simulink model "issue2_drive_demo"  (R2024b)
settings: Solver=FixedStepDiscrete  StartTime=0.0  StopTime=1  FixedStep=.001  RelTol=1e-3
InitFcn:
  | addpath(fullfile(fileparts(get_param(bdroot,'FileName')),'..','matlab'));
model workspace (MAT data in the model file):
  drive_cfg.R = 5.5
  drive_cfg.L = 0.000905
  drive_cfg.psi = 0.00257
  drive_cfg.poles = 7
  drive_cfg.Kt = 0.026985
  drive_cfg.Ts = 0.001
  drive_cfg.delay = 0.000775
  drive_cfg.kp = 0.5
  drive_cfg.ki = 150
  drive_cfg.tracking = 200
  drive_cfg.reference_limit = 0.04
  drive_cfg.voltage_limit = 0.4
  drive_cfg.lsb = 0.0008056640625
settings Model: Creator=Administrator  LastModifiedBy=Administrator

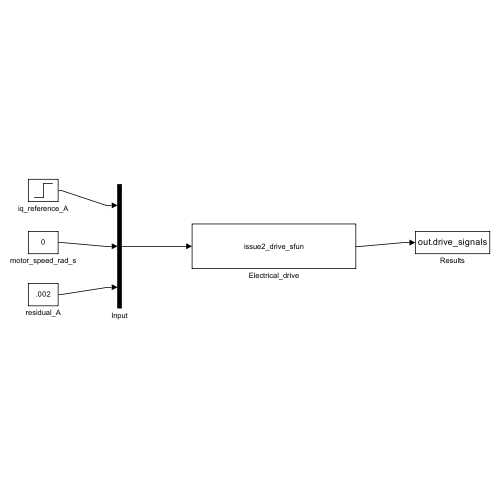
[thumbnail: Simulink's stored preview of the top-level diagram]
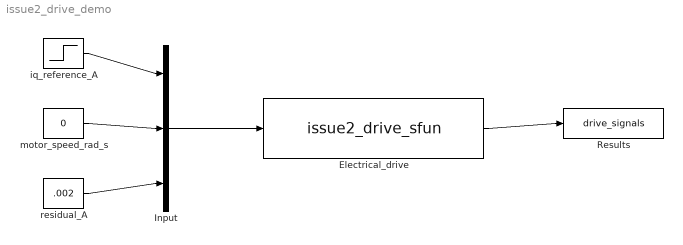
== system issue2_drive_demo ==
  Electrical_drive : M-S-Function  FunctionName=issue2_drive_sfun  Parameters=drive_cfg
  Input : Mux  Inputs=3
  Results : ToWorkspace  VariableName=drive_signals  SaveFormat=Timeseries  SampleTime=-1
  iq_reference_A : Step  Time=.02  After=.02  SampleTime=0
  motor_speed_rad_s : Constant  Value=0
  residual_A : Constant  Value=.002
  wires:
  iq_reference_A/1 -> Input/1
  motor_speed_rad_s/1 -> Input/2
  residual_A/1 -> Input/3
  Input/1 -> Electrical_drive/1
  Electrical_drive/1 -> Results/1
